simulink model "afe_rst_inv_psm_distributed_control_two_delays"  (R2026a)
settings: Solver=ode1be  StopTime=simlength  FixedStep=tc  MaxStep=Tc
values from neighbouring files (symbols this model uses):
  Amplitude_U = 1.16    [grid_fault_generator.m]
  Amplitude_V = Amplitude_U    (= 1.16)    [grid_fault_generator.m]
  Amplitude_W = Amplitude_U    (= 1.16)    [grid_fault_generator.m]
  end_time_LVRT = start_time_LVRT + error_length    [grid_fault_generator.m]
  Igrid_phase_normalization_factor = 270*sqrt(2)    [grid_emulator.m]
  omega_grid_emulator_nom = w_grid    (= 314.159265359)    [grid_emulator.m]
  omega_grid_nom = w_grid    (= 314.159265359)    [grid_emulator.m]
  t_ramp = 20e-3    (= 0.02)    [grid_fault_generator.m]
  ugrid_factor = 1    [grid_emulator.m]
  V_phase_normalization_factor = Vgrid_phase_normalization_factor    [grid_emulator.m]
  Vdc_bez = 1070    [grid_emulator.m]
  Vemu_ref_norm = Vemu_ref * sqrt(2) / V_phase_normalization_factor    [grid_emulator.m]
  vn_eta_pu = 0    [grid_emulator.m]
  vn_xi_pu = 0    [grid_emulator.m]
  vp_xi_pu = 1    [grid_emulator.m]
undefined symbols (not defined in the file or in its folder): Adrso, Aresd, Bresd, CFi, CFu, Cresd, Crso, CTRPIFF_CLIP_RELEASE, dead_time_INV, emf_fb_p, emf_fb_p_ccaller_1, emf_fb_p_ccaller_2, emf_p, emf_p_ccaller_1, emf_p_ccaller_2, fPWM_INV, g0_161Hz, g0_500Hz, g1_161Hz, g1_500Hz, i_grid_neg_eta_lim, i_grid_neg_eta_red_lim, i_grid_neg_xi_lim, i_grid_neg_xi_red_lim, i_grid_pos_eta_lim, i_grid_pos_eta_red_lim, ibez, id_lim, ieta_neg_ref_lim, ieta_pos_ref_lim, iq_lim, ixi_pos_ref_lim, Jm_norm, k_frt_ref, kg, ki_afe, ki_i, ki_id, ki_iq, ki_rc_neg_grid, ki_rc_pos_grid, ki_vs, ki_w, kp_afe, kp_i, kp_id, kp_iq, kp_rc_neg_grid, kp_rc_pos_grid, kp_vs, kp_w, kw, l1, l2, Lalpha_norm, Ld_norm, Ldrso, Lq_norm, Ls_norm, luenberger_l1 ... (+30)
libraries: fl_lib x146, nesl_utility x62, simulink x8, cstblocks_lti x7, sl_discontinuities x3, single_phase_transformer_lib x3, flexshaft_lib x1, permanent_magnet_synchronous_machine x1
(part 2 of 14)

== system afe_rst_inv_psm_distributed_control_two_delays/INV-Modular/threephase_vi_measures ==
  Bus Creator : BusCreator  Inputs=6
  Bus Selector : BusSelector  OutputSignals=usu,usv,usw  OutputAsBus=on
  Bus Selector1 : BusSelector  OutputSignals=isu,iuv,isw  OutputAsBus=on
  Current Sensor : fl_lib/Electrical/Electrical Sensors/Current Sensor
  Current Sensor1 : fl_lib/Electrical/Electrical Sensors/Current Sensor
  Current Sensor2 : fl_lib/Electrical/Electrical Sensors/Current Sensor
  Electrical Reference1 : fl_lib/Electrical/Electrical Elements/Electrical Reference
  Voltage Sensor : fl_lib/Electrical/Electrical Sensors/Voltage Sensor
  Voltage Sensor1 : fl_lib/Electrical/Electrical Sensors/Voltage Sensor
  Voltage Sensor2 : fl_lib/Electrical/Electrical Sensors/Voltage Sensor
  is_uvw/us_uvw : Scope  NumInputPorts=2
      settings: SampleTime=tc  ActiveDisplayYMinimum=-1567.0761  ActiveDisplayYMaximum=1567.45951  DataLoggingVariableName=ScopeData2
  isu_motor : nesl_utility/PS-Simulink Converter  PhysicalDomain=network_engine_domain  SubClassName=ps_output  LeftPortType=input  RightPortType=output  PseudoPeriodic=off  Frequencies=[]  VectorFormat=1-D array  Unit=A  AffineConversion=off
  isv_motor : nesl_utility/PS-Simulink Converter  PhysicalDomain=network_engine_domain  SubClassName=ps_output  LeftPortType=input  RightPortType=output  PseudoPeriodic=off  Frequencies=[]  VectorFormat=1-D array  Unit=A  AffineConversion=off
  isw_motor : nesl_utility/PS-Simulink Converter  PhysicalDomain=network_engine_domain  SubClassName=ps_output  LeftPortType=input  RightPortType=output  PseudoPeriodic=off  Frequencies=[]  VectorFormat=1-D array  Unit=A  AffineConversion=off
  uc_grid : nesl_utility/PS-Simulink Converter  PhysicalDomain=network_engine_domain  SubClassName=ps_output  LeftPortType=input  RightPortType=output  PseudoPeriodic=off  Frequencies=[]  VectorFormat=1-D array  Unit=V  AffineConversion=off
  usu_motor : nesl_utility/PS-Simulink Converter  PhysicalDomain=network_engine_domain  SubClassName=ps_output  LeftPortType=input  RightPortType=output  PseudoPeriodic=off  Frequencies=[]  VectorFormat=1-D array  Unit=V  AffineConversion=off
  usv_motor : nesl_utility/PS-Simulink Converter  PhysicalDomain=network_engine_domain  SubClassName=ps_output  LeftPortType=input  RightPortType=output  PseudoPeriodic=off  Frequencies=[]  VectorFormat=1-D array  Unit=V  AffineConversion=off
  Uu : PMIOPort  Side=Left
  uu : PMIOPort  Port=2  Side=Right
  Uv : PMIOPort  Port=3  Side=Left
  uv : PMIOPort  Port=4  Side=Right
  Uw : PMIOPort  Port=5  Side=Left
  uw : PMIOPort  Port=6  Side=Right
  tag scope: is_uvw_motor=global, us_uvw_motor=global
  wires:
  Bus Creator/1 -> Bus Selector1/1, Bus Selector/1  "vi_data"
  Bus Selector/1 -> [us_uvw_motor]
  isv_motor/1 -> Bus Creator/5  "iuv"
  isu_motor/1 -> Bus Creator/4  "isu"
  isw_motor/1 -> Bus Creator/6  "isw"
  usu_motor/1 -> Bus Creator/1  "usu"
  usv_motor/1 -> Bus Creator/2  "usv"
  uc_grid/1 -> Bus Creator/3  "usw"
  Bus Selector1/1 -> [is_uvw_motor]
  [us_uvw_motor] -> is_uvw/us_uvw/1
  [is_uvw_motor] -> is_uvw/us_uvw/2
  connections:
  Current Sensor1/LConn1 -- Uv/RConn1 -- Voltage Sensor1/LConn1
  Electrical Reference1/LConn1 -- Voltage Sensor/RConn2 -- Voltage Sensor2/RConn2 -- Voltage Sensor1/RConn2
  Voltage Sensor/RConn1 -- usu_motor/LConn1
  Current Sensor/RConn2 -- uu/RConn1
  Voltage Sensor1/RConn1 -- usv_motor/LConn1
  Voltage Sensor2/LConn1 -- Current Sensor2/LConn1 -- Uw/RConn1
  Current Sensor/LConn1 -- Uu/RConn1 -- Voltage Sensor/LConn1
  Current Sensor1/RConn2 -- uv/RConn1
  Voltage Sensor2/RConn1 -- uc_grid/LConn1
  isv_motor/LConn1 -- Current Sensor1/RConn1
  isu_motor/LConn1 -- Current Sensor/RConn1
  isw_motor/LConn1 -- Current Sensor2/RConn1
  Current Sensor2/RConn2 -- uw/RConn1

== system afe_rst_inv_psm_distributed_control_two_delays/brake/switch_5 ==
  Diode : fl_lib/Electrical/Electrical Elements/Diode  Vf=Vgamma V  Ron=Ron Ohm  Goff=1e-8 1/Ohm  i_specify=off  i_priority=None  i=0 A  i_nominal_specify=off  i_nominal_value=1  i_nominal_unit=A  v_specify=off  v_priority=None  v=0 V  v_nominal_specify=off  v_nominal_value=1  v_nominal_unit=V
  Switch : fl_lib/Electrical/Electrical Elements/Switch  R_closed=Ron Ohm  G_open=1e-8 1/Ohm  Threshold=7.5  i_specify=off  i_priority=None  i=0 A  i_nominal_specify=off  i_nominal_value=1  i_nominal_unit=A  v_specify=off  v_priority=None  v=0 V  v_nominal_specify=off  v_nominal_value=1  v_nominal_unit=V
  G : PMIOPort  Side=Left
  C : PMIOPort  Port=2  Side=Left
  E : PMIOPort  Port=3  Side=Right
  connections:
  Switch/RConn2 -- C/RConn1 -- Diode/RConn1
  Switch/RConn1 -- G/RConn1
  Switch/LConn1 -- E/RConn1 -- Diode/LConn1

== system afe_rst_inv_psm_distributed_control_two_delays/brake/switch_6 ==
  Diode : fl_lib/Electrical/Electrical Elements/Diode  Vf=Vgamma V  Ron=Ron Ohm  Goff=1e-8 1/Ohm  i_specify=off  i_priority=None  i=0 A  i_nominal_specify=off  i_nominal_value=1  i_nominal_unit=A  v_specify=off  v_priority=None  v=0 V  v_nominal_specify=off  v_nominal_value=1  v_nominal_unit=V
  C : PMIOPort  Side=Left
  E : PMIOPort  Port=2  Side=Right
  connections:
  E/RConn1 -- Diode/LConn1
  C/RConn1 -- Diode/RConn1

== system afe_rst_inv_psm_distributed_control_two_delays/grid/grid_emulator ==
  3ph_YYg : Subsystem
  Controlled Voltage Source : fl_lib/Electrical/Electrical Sources/Controlled Voltage Source
  Controlled Voltage Source1 : fl_lib/Electrical/Electrical Sources/Controlled Voltage Source
  Controlled Voltage Source2 : fl_lib/Electrical/Electrical Sources/Controlled Voltage Source
  Electrical Reference : fl_lib/Electrical/Electrical Elements/Electrical Reference
  Simulink-PS Converter : nesl_utility/Simulink-PS Converter  PhysicalDomain=network_engine_domain  SubClassName=ps_input  LeftPortType=input  RightPortType=output  PseudoPeriodic=off  Frequencies=[]  NoiseDistribution=none  NoiseParameters=[]  Unit=V  AffineConversion=on  FilteringAndDerivatives=provide  SimscapeFilterOrder=1  InputFilterTimeConstant=0.001  UdotUserProvided=0
  Simulink-PS Converter1 : nesl_utility/Simulink-PS Converter  PhysicalDomain=network_engine_domain  SubClassName=ps_input  LeftPortType=input  RightPortType=output  PseudoPeriodic=off  Frequencies=[]  NoiseDistribution=none  NoiseParameters=[]  Unit=V  AffineConversion=on  FilteringAndDerivatives=provide  SimscapeFilterOrder=1  InputFilterTimeConstant=0.001  UdotUserProvided=0
  Simulink-PS Converter2 : nesl_utility/Simulink-PS Converter  PhysicalDomain=network_engine_domain  SubClassName=ps_input  LeftPortType=input  RightPortType=output  PseudoPeriodic=off  Frequencies=[]  NoiseDistribution=none  NoiseParameters=[]  Unit=V  AffineConversion=on  FilteringAndDerivatives=provide  SimscapeFilterOrder=1  InputFilterTimeConstant=0.001  UdotUserProvided=0
  Solver Configuration : nesl_utility/Solver Configuration  PhysicalDomain=network_engine_domain  SubClassName=solver  LeftPortType=input  RightPortType=generic  Tones=[]  Harmonics=[]  SimulateNoise=off  Profile=off  UseLocalSampling=off  EnableSwitchedLinearOptims=on  FrequencyDomain=off  UseCCode=off  RelTol=0.001  AbsTol=0.001  MinStep=1e-09  ToWorkspace=off  RevertToSquareIcSolve=off  NumHomotopyIterations=100  PhasorMode=off  PhasorModeNumHarmonics=1  ConsistencySolver=NEWTON_FTOL  CanonicalOrdering=UNORDERED  OptimizeIntermediates=UNOPTIMIZED  IndexReductionMethod=DerivativeReplacement  DoDC=off  ResidualTolerance=1e-09  ConsistencyTolSource=GLOBAL  ConsistencyAbsTol=0.001  ConsistencyRelTol=0.001  ConsistencyTolFactor=0.001  UseLocalSolver=on  LocalSolverChoice=NE_BACKWARD_EULER_ADVANCER  ResolveIndetEquations=on  FunctionEvalNumThread=1  LocalSolverSampleTime=tc  DoFixedCost=on  MaxNonlinIter=3  MaxModeIter=2  ComputeImpulses=off  ImpulseIterations=2  LinearAlgebra=auto  LinearAlgebraNumThread=0  EquationFormulation=NE_TIME_EF  DelaysMemoryBudget=1024  AutomaticFiltering=on  FilteringTimeConstant=0.001  PartitionStorageMethod=AS_NEEDED  PartitionMemoryBudget=1024  PartitionMethod=ROBUST  MultibodyUseLocalSolver=off  MultibodyLocalSolverChoice=ODE1  MultibodyLocalSolverSampleTime=0.001
  grid_emulator : Subsystem
  threephase_vi_measures : Subsystem
  u1 : PMIOPort  Side=Right
  u2 : PMIOPort  Port=2  Side=Right
  u3 : PMIOPort  Port=3  Side=Right
  wires:
  grid_emulator/2(Vmb) -> Simulink-PS Converter1/1
  grid_emulator/3(Vmc) -> Simulink-PS Converter2/1
  grid_emulator/1(Vma) -> Simulink-PS Converter/1
  connections:
  Simulink-PS Converter/RConn1 -- Controlled Voltage Source/RConn1
  Simulink-PS Converter1/RConn1 -- Controlled Voltage Source1/RConn1
  Simulink-PS Converter2/RConn1 -- Controlled Voltage Source2/RConn1
  Electrical Reference/LConn1 -- Solver Configuration/RConn1 -- Controlled Voltage Source/RConn2 -- Controlled Voltage Source1/RConn2 -- Controlled Voltage Source2/RConn2
  3ph_YYg/RConn1 -- u1/RConn1
  3ph_YYg/RConn2 -- u2/RConn1
  3ph_YYg/RConn3 -- u3/RConn1
  threephase_vi_measures/LConn1 -- Controlled Voltage Source/LConn1
  threephase_vi_measures/LConn2 -- Controlled Voltage Source1/LConn1
  threephase_vi_measures/LConn3 -- Controlled Voltage Source2/LConn1
  threephase_vi_measures/RConn1 -- 3ph_YYg/LConn1
  threephase_vi_measures/RConn2 -- 3ph_YYg/LConn2
  threephase_vi_measures/RConn3 -- 3ph_YYg/LConn3

== system afe_rst_inv_psm_distributed_control_two_delays/grid/instantaneus_power ==
  Vline : Inport
  Iline : Inport  Port=2
  Demux2 : Demux  Outputs=3
  Demux3 : Demux  Outputs=3
  Fcn1 : Fcn  Expr=u(1)/(sqrt(u(1)^2+u(2)^2))
  Gain2 : Gain  Gain=3/2
  Gain3 : Gain  Gain=3/2
  Mux1 : Mux  Inputs=2
  Product{,1..3} (4 alike) : Product  RndMeth=Zero
  Sum : Sum  Inputs=|++
  Sum1 : Sum  Inputs=|+-
  To Workspace1 : ToWorkspace  VariableName=va_line_rms_sim  SampleTime=ts_afe
      settings: MaxDataPoints=Ns_afe
  To Workspace2 : ToWorkspace  VariableName=vb_line_rms_sim  SampleTime=ts_afe
      settings: MaxDataPoints=Ns_afe
  To Workspace3 : ToWorkspace  VariableName=vc_line_rms_sim  SampleTime=ts_afe
      settings: MaxDataPoints=Ns_afe
  To Workspace4 : ToWorkspace  VariableName=ia_line_rms_sim  SampleTime=ts_afe
      settings: MaxDataPoints=Ns_afe
  To Workspace5 : ToWorkspace  VariableName=ib_line_rms_sim  SampleTime=ts_afe
      settings: MaxDataPoints=Ns_afe
  To Workspace6 : ToWorkspace  VariableName=ic_line_rms_sim  SampleTime=ts_afe
      settings: MaxDataPoints=Ns_afe
  To Workspace7 : ToWorkspace  VariableName=Pline_avg_sim  SampleTime=ts_afe
      settings: MaxDataPoints=Ns_afe
  To Workspace8 : ToWorkspace  VariableName=Qline_avg_sim  SampleTime=ts_afe
      settings: MaxDataPoints=Ns_afe
  abc2alphabeta : Subsystem
  "abc2alphabeta " : Subsystem
  moving_avarage : Subsystem
  moving_avarage1 : Subsystem
  rms : Subsystem
  rms1 : Subsystem
  rms2 : Subsystem
  rms3 : Subsystem
  rms4 : Subsystem
  rms5 : Subsystem
  tag scope: Pline_avg=global, Qline_avg=global, cos_phi_avg=global
  wires:
  Gain3/1 -> moving_avarage1/1(In), To Workspace8/1
  Gain2/1 -> moving_avarage/1(In), To Workspace7/1
  Demux2/1 -> abc2alphabeta/1(a), rms/1(In1)
  Vline/1 -> Demux2/1
  Iline/1 -> Demux3/1
  abc2alphabeta/2(vline_beta) -> Product1/1, Product2/1
  "abc2alphabeta "/2(i_line_beta) -> Product3/1, Product1/2
  abc2alphabeta/1(vline_alpha) -> Product/1, Product3/2
  "abc2alphabeta "/1(i_line_alpha) -> Product2/2, Product/2
  Product/1 -> Sum/1
  Product1/1 -> Sum/2
  Product2/1 -> Sum1/1
  Product3/1 -> Sum1/2
  Sum1/1 -> Gain3/1
  Sum/1 -> Gain2/1
  Demux2/2 -> abc2alphabeta/2(b), rms1/1(In1)
  Demux2/3 -> abc2alphabeta/3(c), rms2/1(In1)
  Demux3/1 -> "abc2alphabeta "/1(a), rms3/1(In1)
  Demux3/2 -> "abc2alphabeta "/2(b), rms4/1(In1)
  Demux3/3 -> rms5/1(In1), "abc2alphabeta "/3(c)
  moving_avarage/1(Mean) -> [Pline_avg]
  moving_avarage1/1(Mean) -> [Qline_avg]
  [Qline_avg] -> Mux1/2
  Mux1/1 -> Fcn1/1
  Fcn1/1 -> [cos_phi_avg]
  [Pline_avg] -> Mux1/1
  rms/1(Out1) -> To Workspace1/1
  rms2/1(Out1) -> To Workspace3/1
  rms1/1(Out1) -> To Workspace2/1
  rms5/1(Out1) -> To Workspace6/1
  rms4/1(Out1) -> To Workspace5/1
  rms3/1(Out1) -> To Workspace4/1

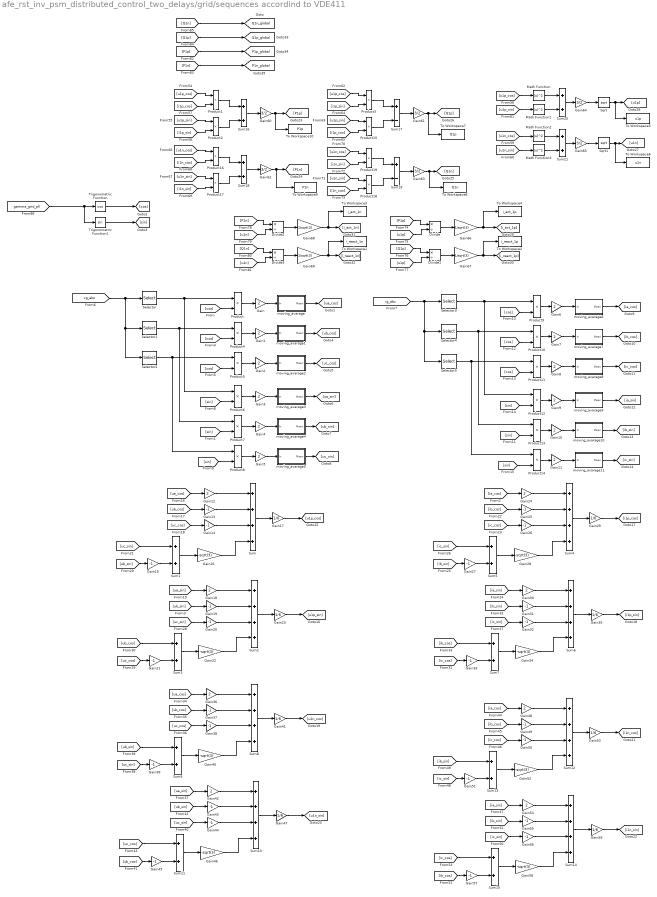
== system afe_rst_inv_psm_distributed_control_two_delays/grid/sequences accordind to VDE411 ==
  Divide{,1..3} (4 alike) : Product  Inputs=*/
  Gain{,1..12,18,24,30,36,42,48,54} (20 alike) : Gain  Gain=2
  Gain{13..15,19..21,25..27,31..33,37..39,43..45,49..51,55..57} (24 alike) : Gain  Gain=-1
  Gain{16,22,28,34,40,46,52,58} (8 alike) : Gain  Gain=-sqrt(3)
  Gain{17,23,29,35,41,47,53,59} (8 alike) : Gain  Gain=1/6
  Gain{60..65} (6 alike) : Gain  Gain=3/2
  Gain{66..69} (4 alike) : Gain  Gain=1/sqrt(3)
  Math Function{,1..3} (4 alike) : Math  Operator=magnitude^2  SignedPower=on
  Product{,1..19} (20 alike) : Product  RndMeth=Zero
  Selector : Selector  InputPortWidth=3  IndexOptions=Index vector (dialog)  Indices=1  OutputSizes=1
  Selector1 : Selector  InputPortWidth=3  IndexOptions=Index vector (dialog)  Indices=2  OutputSizes=1
  Selector2 : Selector  InputPortWidth=3  IndexOptions=Index vector (dialog)  Indices=3  OutputSizes=1
  Selector3 : Selector  InputPortWidth=3  IndexOptions=Index vector (dialog)  Indices=1  OutputSizes=1
  Selector4 : Selector  InputPortWidth=3  IndexOptions=Index vector (dialog)  Indices=2  OutputSizes=1
  Selector5 : Selector  InputPortWidth=3  IndexOptions=Index vector (dialog)  Indices=3  OutputSizes=1
  Sqrt : Sqrt
  Sqrt1 : Sqrt
  Sum{,2,4,6,8,10,12,14} (8 alike) : Sum  Inputs=++++
  Sum{1,3,5,7,9,11,13,15..16,18,20..21} (12 alike) : Sum
  Sum17 : Sum  Inputs=+-
  Sum19 : Sum  Inputs=+-
  To Workspace1 : ToWorkspace  VariableName=i_react_1n  SampleTime=ts_afe
      settings: MaxDataPoints=Ns_afe
  To Workspace10 : ToWorkspace  VariableName=P1p  SampleTime=ts_afe
      settings: MaxDataPoints=Ns_afe
  To Workspace2 : ToWorkspace  VariableName=i_react_1p  SampleTime=ts_afe
      settings: MaxDataPoints=Ns_afe
  To Workspace3 : ToWorkspace  VariableName=i_act_1n  SampleTime=ts_afe
      settings: MaxDataPoints=Ns_afe
  To Workspace4 : ToWorkspace  VariableName=i_act_1p  SampleTime=ts_afe
      settings: MaxDataPoints=Ns_afe
  To Workspace5 : ToWorkspace  VariableName=u1p  SampleTime=ts_afe
      settings: MaxDataPoints=Ns_afe
  To Workspace6 : ToWorkspace  VariableName=u1n  SampleTime=ts_afe
      settings: MaxDataPoints=Ns_afe
  To Workspace7 : ToWorkspace  VariableName=Q1p  SampleTime=ts_afe
      settings: MaxDataPoints=Ns_afe
  To Workspace8 : ToWorkspace  VariableName=Q1n  SampleTime=ts_afe
      settings: MaxDataPoints=Ns_afe
  To Workspace9 : ToWorkspace  VariableName=P1n  SampleTime=ts_afe
      settings: MaxDataPoints=Ns_afe
  Trigonometric Function : Trigonometry  Operator=cos
  Trigonometric Function1 : Trigonometry
  moving_avarage : Subsystem
  moving_avarage1 : Subsystem
  moving_avarage10 : Subsystem
  moving_avarage11 : Subsystem
  moving_avarage2 : Subsystem
  moving_avarage3 : Subsystem
  moving_avarage4 : Subsystem
  moving_avarage5 : Subsystem
  moving_avarage6 : Subsystem
  moving_avarage7 : Subsystem
  moving_avarage8 : Subsystem
  moving_avarage9 : Subsystem
  tag scope: P1n_global=global, P1p_global=global, Q1n_global=global, Q1p_global=global
  wires:
  [vg_abc] -> Selector2/1, Selector1/1, Selector/1
  Trigonometric Function1/1 -> [sin]
  Trigonometric Function/1 -> [cos]
  [gamma_grid_pll] -> Trigonometric Function/1, Trigonometric Function1/1
  [cos] -> Product/2
  Product/1 -> Gain/1
  [cos] -> Product4/2
  Product4/1 -> Gain1/1
  [cos] -> Product5/2
  Product5/1 -> Gain2/1
  [sin] -> Product6/2
  Selector/1 -> Product6/1, Product/1
  Product6/1 -> Gain3/1
  [sin] -> Product7/2
  Selector1/1 -> Product7/1, Product4/1
  Product7/1 -> Gain4/1
  [sin] -> Product8/2
  Selector2/1 -> Product8/1, Product5/1
  Product8/1 -> Gain5/1
  [ig_abc] -> Selector3/1, Selector4/1, Selector5/1
  [cos] -> Product9/2
  Product9/1 -> Gain6/1
  [cos] -> Product10/2
  Product10/1 -> Gain7/1
  [cos] -> Product11/2
  Product11/1 -> Gain8/1
  [sin] -> Product12/2
  Selector3/1 -> Product9/1, Product12/1
  Product12/1 -> Gain9/1
  [sin] -> Product13/2
  Selector4/1 -> Product10/1, Product13/1
  Product13/1 -> Gain10/1
  [sin] -> Product14/2
  Selector5/1 -> Product11/1, Product14/1
  Product14/1 -> Gain11/1
  Gain/1 -> moving_avarage/1(In)
  moving_avarage/1(Mean) -> [ua_cos]
  Gain1/1 -> moving_avarage1/1(In)
  Gain2/1 -> moving_avarage2/1(In)
  Gain3/1 -> moving_avarage3/1(In)
  Gain4/1 -> moving_avarage4/1(In)
  Gain5/1 -> moving_avarage5/1(In)
  Gain6/1 -> moving_avarage6/1(In)
  Gain7/1 -> moving_avarage7/1(In)
  Gain8/1 -> moving_avarage8/1(In)
  Gain9/1 -> moving_avarage9/1(In)
  Gain10/1 -> moving_avarage10/1(In)
  Gain11/1 -> moving_avarage11/1(In)
  [ua_cos] -> Gain12/1
  [ub_cos] -> Gain13/1
  [uc_cos] -> Gain14/1
  [uc_sin] -> Sum1/1
  Gain15/1 -> Sum1/2
  [ub_sin] -> Gain15/1
  Sum1/1 -> Gain16/1
  Gain16/1 -> Sum/4
  Gain14/1 -> Sum/3
  Gain13/1 -> Sum/2
  Gain12/1 -> Sum/1
  Sum/1 -> Gain17/1
  Gain17/1 -> [u1p_cos]
  [ua_sin] -> Gain18/1
  [ub_sin] -> Gain19/1
  [uc_sin] -> Gain20/1
  [ub_cos] -> Sum3/1
  Gain21/1 -> Sum3/2
  [uc_cos] -> Gain21/1
  Sum3/1 -> Gain22/1
  Gain22/1 -> Sum2/4
  Gain20/1 -> Sum2/3
  Gain19/1 -> Sum2/2
  Gain18/1 -> Sum2/1
  Sum2/1 -> Gain23/1
  Gain23/1 -> [u1p_sin]
  [ia_cos] -> Gain24/1
  [ib_cos] -> Gain25/1
  [ic_cos] -> Gain26/1
  [ic_sin] -> Sum5/1
  Gain27/1 -> Sum5/2
  [ib_sin] -> Gain27/1
  Sum5/1 -> Gain28/1
  Gain28/1 -> Sum4/4
  Gain26/1 -> Sum4/3
  Gain25/1 -> Sum4/2
  Gain24/1 -> Sum4/1
  Sum4/1 -> Gain29/1
  Gain29/1 -> [i1p_cos]
  [ia_sin] -> Gain30/1
  [ib_sin] -> Gain31/1
  [ic_sin] -> Gain32/1
  [ib_cos] -> Sum7/1
  Gain33/1 -> Sum7/2
  [ic_cos] -> Gain33/1
  Sum7/1 -> Gain34/1
  Gain34/1 -> Sum6/4
  Gain32/1 -> Sum6/3
  Gain31/1 -> Sum6/2
  Gain30/1 -> Sum6/1
  Sum6/1 -> Gain35/1
  Gain35/1 -> [i1p_sin]
  [ua_cos] -> Gain36/1
  [ub_cos] -> Gain37/1
  [uc_cos] -> Gain38/1
  [ub_sin] -> Sum9/1
  Gain39/1 -> Sum9/2
  [uc_sin] -> Gain39/1
  Sum9/1 -> Gain40/1
  Gain40/1 -> Sum8/4
  Gain38/1 -> Sum8/3
  Gain37/1 -> Sum8/2
  Gain36/1 -> Sum8/1
  Sum8/1 -> Gain41/1
  Gain41/1 -> [u1n_cos]
  [ua_sin] -> Gain42/1
  [ub_sin] -> Gain43/1
  [uc_sin] -> Gain44/1
  [uc_cos] -> Sum11/1
  Gain45/1 -> Sum11/2
  [ub_cos] -> Gain45/1
  Sum11/1 -> Gain46/1
  Gain46/1 -> Sum10/4
  Gain44/1 -> Sum10/3
  Gain43/1 -> Sum10/2
  Gain42/1 -> Sum10/1
  Sum10/1 -> Gain47/1
  Gain47/1 -> [u1n_sin]
  [ia_cos] -> Gain48/1
  [ib_cos] -> Gain49/1
  [ic_cos] -> Gain50/1
  [ib_sin] -> Sum13/1
  Gain51/1 -> Sum13/2
  [ic_sin] -> Gain51/1
  Sum13/1 -> Gain52/1
  Gain52/1 -> Sum12/4
  Gain50/1 -> Sum12/3
  Gain49/1 -> Sum12/2
  Gain48/1 -> Sum12/1
  Sum12/1 -> Gain53/1
  Gain53/1 -> [i1n_cos]
  [ia_sin] -> Gain54/1
  [ib_sin] -> Gain55/1
  [ic_sin] -> Gain56/1
  [ic_cos] -> Sum15/1
  Gain57/1 -> Sum15/2
  [ib_cos] -> Gain57/1
  Sum15/1 -> Gain58/1
  Gain58/1 -> Sum14/4
  Gain56/1 -> Sum14/3
  Gain55/1 -> Sum14/2
  Gain54/1 -> Sum14/1
  Sum14/1 -> Gain59/1
  Gain59/1 -> [i1n_sin]
  Sum16/1 -> Gain60/1
  Product1/1 -> Sum16/1
  Product2/1 -> Sum16/2
  Gain60/1 -> To Workspace10/1, [P1p]
  [u1p_cos] -> Product1/1
  [i1p_cos] -> Product1/2
  [u1p_sin] -> Product2/1
  [i1p_sin] -> Product2/2
  Sum17/1 -> Gain61/1
  Product3/1 -> Sum17/1
  Product15/1 -> Sum17/2
  Gain61/1 -> To Workspace7/1, [Q1p]
  [u1p_cos] -> Product3/1
  [i1p_sin] -> Product3/2
  [u1p_sin] -> Product15/1
  [i1p_cos] -> Product15/2
  Sum18/1 -> Gain62/1
  Product16/1 -> Sum18/1
  Product17/1 -> Sum18/2
  Gain62/1 -> To Workspace9/1, [P1n]
  [u1n_cos] -> Product16/1
  [i1n_cos] -> Product16/2
  [u1n_sin] -> Product17/1
  [i1n_sin] -> Product17/2
  Sum19/1 -> Gain63/1
  Product19/1 -> Sum19/1
  Product18/1 -> Sum19/2
  Gain63/1 -> To Workspace8/1, [Q1n]
  [u1n_cos] -> Product19/1
  [i1n_sin] -> Product19/2
  [u1n_sin] -> Product18/1
  [i1n_cos] -> Product18/2
  [u1p_cos] -> Math Function/1
  [u1p_sin] -> Math Function1/1
  Math Function/1 -> Sum20/1
  Math Function1/1 -> Sum20/2
  Sum20/1 -> Gain64/1
  Gain64/1 -> Sqrt/1
  Sqrt/1 -> To Workspace5/1, [u1p]
  [u1n_cos] -> Math Function2/1
  [u1n_sin] -> Math Function3/1
  Math Function2/1 -> Sum21/1
  Math Function3/1 -> Sum21/2
  Sum21/1 -> Gain65/1
  Gain65/1 -> Sqrt1/1
  Sqrt1/1 -> To Workspace6/1, [u1n]
  [P1p] -> Divide/1
  [u1p] -> Divide/2
  Divide/1 -> Gain66/1
  Gain66/1 -> To Workspace4/1, [i_act_1p]
  [Q1p] -> Divide1/1
  [u1p] -> Divide1/2
  Divide1/1 -> Gain67/1
  Gain67/1 -> To Workspace2/1, [i_react_1p]
  [P1n] -> Divide2/1
  [u1n] -> Divide2/2
  Divide2/1 -> Gain68/1
  Gain68/1 -> To Workspace3/1, [i_act_1n]
  [Q1n] -> Divide3/1
  [u1n] -> Divide3/2
  Divide3/1 -> Gain69/1
  Gain69/1 -> To Workspace1/1, [i_react_1n]
  moving_avarage1/1(Mean) -> [ub_cos]
  moving_avarage2/1(Mean) -> [uc_cos]
  moving_avarage3/1(Mean) -> [ua_sin]
  moving_avarage4/1(Mean) -> [ub_sin]
  moving_avarage5/1(Mean) -> [uc_sin]
  moving_avarage6/1(Mean) -> [ia_cos]
  moving_avarage7/1(Mean) -> [ib_cos]
  moving_avarage8/1(Mean) -> [ic_cos]
  moving_avarage9/1(Mean) -> [ia_sin]
  moving_avarage10/1(Mean) -> [ib_sin]
  moving_avarage11/1(Mean) -> [ic_sin]
  [Q1n] -> [Q1n_global]
  [Q1p] -> [Q1p_global]
  [P1p] -> [P1p_global]
  [P1n] -> [P1n_global]

== system afe_rst_inv_psm_distributed_control_two_delays/grid/threephase_vi_measures ==
  Bus Creator : BusCreator  Inputs=6
  Bus Selector : BusSelector  OutputSignals=ua,ub,uc  OutputAsBus=on
  Bus Selector1 : BusSelector  OutputSignals=iga,igb,igc  OutputAsBus=on
  Current Sensor : fl_lib/Electrical/Electrical Sensors/Current Sensor
  Current Sensor1 : fl_lib/Electrical/Electrical Sensors/Current Sensor
  Current Sensor2 : fl_lib/Electrical/Electrical Sensors/Current Sensor
  Electrical Reference1 : fl_lib/Electrical/Electrical Elements/Electrical Reference
  Voltage Sensor : fl_lib/Electrical/Electrical Sensors/Voltage Sensor
  Voltage Sensor1 : fl_lib/Electrical/Electrical Sensors/Voltage Sensor
  Voltage Sensor2 : fl_lib/Electrical/Electrical Sensors/Voltage Sensor
  ia_grid : nesl_utility/PS-Simulink Converter  PhysicalDomain=network_engine_domain  SubClassName=ps_output  LeftPortType=input  RightPortType=output  PseudoPeriodic=off  Frequencies=[]  VectorFormat=1-D array  Unit=A  AffineConversion=off
  ib_grid : nesl_utility/PS-Simulink Converter  PhysicalDomain=network_engine_domain  SubClassName=ps_output  LeftPortType=input  RightPortType=output  PseudoPeriodic=off  Frequencies=[]  VectorFormat=1-D array  Unit=A  AffineConversion=off
  ic_grid : nesl_utility/PS-Simulink Converter  PhysicalDomain=network_engine_domain  SubClassName=ps_output  LeftPortType=input  RightPortType=output  PseudoPeriodic=off  Frequencies=[]  VectorFormat=1-D array  Unit=A  AffineConversion=off
  ig_abc/ug_abc : Scope  NumInputPorts=2
      settings: SampleTime=tc  ActiveDisplayYMinimum=-781.63744  ActiveDisplayYMaximum=887.15685  DataLoggingVariableName=ScopeData2
  ua_grid : nesl_utility/PS-Simulink Converter  PhysicalDomain=network_engine_domain  SubClassName=ps_output  LeftPortType=input  RightPortType=output  PseudoPeriodic=off  Frequencies=[]  VectorFormat=1-D array  Unit=V  AffineConversion=off
  ub_grid : nesl_utility/PS-Simulink Converter  PhysicalDomain=network_engine_domain  SubClassName=ps_output  LeftPortType=input  RightPortType=output  PseudoPeriodic=off  Frequencies=[]  VectorFormat=1-D array  Unit=V  AffineConversion=off
  uc_grid : nesl_utility/PS-Simulink Converter  PhysicalDomain=network_engine_domain  SubClassName=ps_output  LeftPortType=input  RightPortType=output  PseudoPeriodic=off  Frequencies=[]  VectorFormat=1-D array  Unit=V  AffineConversion=off
  Ua : PMIOPort  Side=Left
  ua : PMIOPort  Port=2  Side=Right
  Ub : PMIOPort  Port=3  Side=Left
  ub : PMIOPort  Port=4  Side=Right
  Uc : PMIOPort  Port=5  Side=Left
  uc : PMIOPort  Port=6  Side=Right
  tag scope: ig_abc=global, vg_abc=global
  wires:
  Bus Creator/1 -> Bus Selector1/1, Bus Selector/1  "vi_data"
  Bus Selector/1 -> [vg_abc]
  ib_grid/1 -> Bus Creator/5  "igb"
  ia_grid/1 -> Bus Creator/4  "iga"
  ic_grid/1 -> Bus Creator/6  "igc"
  ua_grid/1 -> Bus Creator/1  "ua"
  ub_grid/1 -> Bus Creator/2  "ub"
  uc_grid/1 -> Bus Creator/3  "uc"
  Bus Selector1/1 -> [ig_abc]
  [vg_abc] -> ig_abc/ug_abc/2
  [ig_abc] -> ig_abc/ug_abc/1
  connections:
  Current Sensor1/LConn1 -- ub/RConn1 -- Voltage Sensor1/LConn1
  Electrical Reference1/LConn1 -- Voltage Sensor/RConn2 -- Voltage Sensor2/RConn2 -- Voltage Sensor1/RConn2
  Voltage Sensor/RConn1 -- ua_grid/LConn1
  Ua/RConn1 -- Current Sensor/RConn2
  Voltage Sensor1/RConn1 -- ub_grid/LConn1
  Voltage Sensor2/LConn1 -- uc/RConn1 -- Current Sensor2/LConn1
  Current Sensor/LConn1 -- ua/RConn1 -- Voltage Sensor/LConn1
  Ub/RConn1 -- Current Sensor1/RConn2
  Voltage Sensor2/RConn1 -- uc_grid/LConn1
  ib_grid/LConn1 -- Current Sensor1/RConn1
  ia_grid/LConn1 -- Current Sensor/RConn1
  ic_grid/LConn1 -- Current Sensor2/RConn1
  Uc/RConn1 -- Current Sensor2/RConn2

== system afe_rst_inv_psm_distributed_control_two_delays/grid filter/threephase_vi_measures_stack ==
  Bus Creator : BusCreator  Inputs=6
  Current Sensor : fl_lib/Electrical/Electrical Sensors/Current Sensor
  Current Sensor1 : fl_lib/Electrical/Electrical Sensors/Current Sensor
  Current Sensor2 : fl_lib/Electrical/Electrical Sensors/Current Sensor
  Electrical Reference1 : fl_lib/Electrical/Electrical Elements/Electrical Reference
  Selector : Selector  InputPortWidth=6  IndexOptions=Index vector (dialog)  Indices=[1 2 3]  OutputSizes=1
  Selector1 : Selector  InputPortWidth=6  IndexOptions=Index vector (dialog)  Indices=[4 5 6]  OutputSizes=1
  Voltage Sensor : fl_lib/Electrical/Electrical Sensors/Voltage Sensor
  Voltage Sensor1 : fl_lib/Electrical/Electrical Sensors/Voltage Sensor
  Voltage Sensor2 : fl_lib/Electrical/Electrical Sensors/Voltage Sensor
  ia_afe : nesl_utility/PS-Simulink Converter  PhysicalDomain=network_engine_domain  SubClassName=ps_output  LeftPortType=input  RightPortType=output  PseudoPeriodic=off  Frequencies=[]  VectorFormat=1-D array  Unit=A  AffineConversion=off
  ib_afe : nesl_utility/PS-Simulink Converter  PhysicalDomain=network_engine_domain  SubClassName=ps_output  LeftPortType=input  RightPortType=output  PseudoPeriodic=off  Frequencies=[]  VectorFormat=1-D array  Unit=A  AffineConversion=off
  ic_afe : nesl_utility/PS-Simulink Converter  PhysicalDomain=network_engine_domain  SubClassName=ps_output  LeftPortType=input  RightPortType=output  PseudoPeriodic=off  Frequencies=[]  VectorFormat=1-D array  Unit=A  AffineConversion=off
  is_abc/us_abc : Scope  NumInputPorts=2
      settings: SampleTime=tc  ActiveDisplayYMinimum=-168.28271  ActiveDisplayYMaximum=145.46709
  ua_afe : nesl_utility/PS-Simulink Converter  PhysicalDomain=network_engine_domain  SubClassName=ps_output  LeftPortType=input  RightPortType=output  PseudoPeriodic=off  Frequencies=[]  VectorFormat=1-D array  Unit=V  AffineConversion=off
  ub_afe : nesl_utility/PS-Simulink Converter  PhysicalDomain=network_engine_domain  SubClassName=ps_output  LeftPortType=input  RightPortType=output  PseudoPeriodic=off  Frequencies=[]  VectorFormat=1-D array  Unit=V  AffineConversion=off
  uc_afe : nesl_utility/PS-Simulink Converter  PhysicalDomain=network_engine_domain  SubClassName=ps_output  LeftPortType=input  RightPortType=output  PseudoPeriodic=off  Frequencies=[]  VectorFormat=1-D array  Unit=V  AffineConversion=off
  Ua : PMIOPort  Side=Left
  ua : PMIOPort  Port=2  Side=Right
  Ub : PMIOPort  Port=3  Side=Left
  ub : PMIOPort  Port=4  Side=Right
  Uc : PMIOPort  Port=5  Side=Left
  uc : PMIOPort  Port=6  Side=Right
  tag scope: is_abc=global, vs_abc=global
  wires:
  Bus Creator/1 -> Selector1/1, Selector/1  "vi_data"
  Selector/1 -> [vs_abc]
  ib_afe/1 -> Bus Creator/5  "ib_afe"
  ia_afe/1 -> Bus Creator/4  "ia_afe"
  ic_afe/1 -> Bus Creator/6  "ic_afe"
  ua_afe/1 -> Bus Creator/1  "ua_afe"
  ub_afe/1 -> Bus Creator/2  "ub_afe"
  uc_afe/1 -> Bus Creator/3  "uc_afe"
  Selector1/1 -> [is_abc]
  [is_abc] -> is_abc/us_abc/1
  [vs_abc] -> is_abc/us_abc/2
  connections:
  Current Sensor1/LConn1 -- Voltage Sensor1/LConn1 -- Ub/RConn1
  Electrical Reference1/LConn1 -- Voltage Sensor1/RConn2 -- Voltage Sensor2/RConn2 -- Voltage Sensor/RConn2
  Voltage Sensor/RConn1 -- ua_afe/LConn1
  Current Sensor/RConn2 -- ua/RConn1
  Voltage Sensor1/RConn1 -- ub_afe/LConn1
  Voltage Sensor2/LConn1 -- Uc/RConn1 -- Current Sensor2/LConn1
  Current Sensor/LConn1 -- Voltage Sensor/LConn1 -- Ua/RConn1
  Current Sensor1/RConn2 -- ub/RConn1
  Voltage Sensor2/RConn1 -- uc_afe/LConn1
  ib_afe/LConn1 -- Current Sensor1/RConn1
  ia_afe/LConn1 -- Current Sensor/RConn1
  ic_afe/LConn1 -- Current Sensor2/RConn1
  Current Sensor2/RConn2 -- uc/RConn1

== system afe_rst_inv_psm_distributed_control_two_delays/mainboard_afe/current_sequence_avg ==
  i_grid_pos_xi : Inport
  i_grid_pos_eta : Inport  Port=2
  i_grid_neg_xi : Inport  Port=3
  i_grid_neg_eta : Inport  Port=4
  Moving Average Filter5 : Subsystem
  Moving Average Filter6 : Subsystem
  Moving Average Filter7 : Subsystem
  Moving Average Filter8 : Subsystem
  i_grid_pos_xi_avg : Outport
  i_grid_pos_eta_avg : Outport  Port=2
  i_grid_neg_xi_avg : Outport  Port=3
  i_grid_neg_eta_avg : Outport  Port=4
  wires:
  [omega_grid_pll] -> Moving Average Filter5/2(In3), Moving Average Filter6/2(In3), Moving Average Filter7/2(In3), Moving Average Filter8/2(In3)
  Moving Average Filter8/1(xi) -> i_grid_neg_eta_avg/1
  i_grid_neg_eta/1 -> Moving Average Filter8/1(In2)
  i_grid_neg_xi/1 -> Moving Average Filter7/1(In2)
  Moving Average Filter7/1(xi) -> i_grid_neg_xi_avg/1
  Moving Average Filter6/1(xi) -> i_grid_pos_eta_avg/1
  i_grid_pos_eta/1 -> Moving Average Filter6/1(In2)
  i_grid_pos_xi/1 -> Moving Average Filter5/1(In2)
  Moving Average Filter5/1(xi) -> i_grid_pos_xi_avg/1

== system afe_rst_inv_psm_distributed_control_two_delays/mainboard_afe/dq_pll ==
  note: SRF-PLL
  phase_pll/phase_grid : Scope  NumInputPorts=2
      settings: SampleTime=ts_afe  ActiveDisplayYMinimum=-3.92699  ActiveDisplayYMaximum=3.92699
  pll_stageA : Subsystem
  pll_stageB : Subsystem
  tag scope: gamma_grid_pll=global
  wires:
  pll_stageB/1(gamma_grid_pll) -> pll_stageA/1(gamma_grid), phase_pll/phase_grid/1, [gamma_grid_pll]
  pll_stageA/2(u_grid_pos_eta) -> pll_stageB/2(u_grid_pos_eta)  "u_grid_pos_eta"
  pll_stageA/1(u_grid_pos_xi) -> pll_stageB/1(u_grid_pos_xi)  "u_grid_pos_xi"
  [gamma_grid_emulator] -> phase_pll/phase_grid/2

== system afe_rst_inv_psm_distributed_control_two_delays/mainboard_afe/grid_current_sampling_and_alpha_beta_transformation ==
  Mux : Mux  Inputs=3
  Selector : Selector  InputPortWidth=3  IndexOptions=Index vector (dialog)  Indices=1  OutputSizes=1
  i_abc2alphabeta : MATLAB Function  TreatAsAtomicUnit=on  SystemSampleTime=ts_afe
  ig_hat/ig : Scope  NumInputPorts=2
      settings: SampleTime=tc  ActiveDisplayYMinimum=-1.06426  ActiveDisplayYMaximum=1.44682  DataLoggingVariableName=ScopeData2
  ig_hat/ig1 : Scope  NumInputPorts=2
      settings: SampleTime=tc  ActiveDisplayYMinimum=-2.36968  ActiveDisplayYMaximum=2.03597  DataLoggingVariableName=ScopeData3
  iga_measure : Subsystem
  i_grid_alpha : Outport
  i_grid_beta : Outport  Port=2
  wires:
  i_abc2alphabeta/2(beta) -> i_grid_beta/1  "i_grid_beta"
  i_abc2alphabeta/1(alpha) -> i_grid_alpha/1  "i_grid_alpha"
  [ig_abc] -> iga_measure/1(ig)
  [iga_pu_dba_fb_mbafe] -> Mux/1
  [igb_pu_dbb_fb_mbafe] -> Mux/2
  [igc_pu_dbc_fb_mbafe] -> Mux/3
  Mux/1 -> ig_hat/ig1/1
  iga_measure/1(ig_pu) -> i_abc2alphabeta/1(i_abc), Selector/1, ig_hat/ig1/2
  [iga_pu_dba] -> ig_hat/ig/1
  Selector/1 -> ig_hat/ig/2

== system afe_rst_inv_psm_distributed_control_two_delays/mainboard_afe/grid_voltage_sampling_and_alpha_beta_transformation ==
  Mux : Mux  Inputs=3
  v_abc2alphabeta : MATLAB Function  TreatAsAtomicUnit=on  SystemSampleTime=ts_afe
  u_grid_alpha : Outport
  u_grid_beta : Outport  Port=2
  wires:
  v_abc2alphabeta/1(alpha) -> u_grid_alpha/1  "u_grid_alpha"
  v_abc2alphabeta/2(beta) -> u_grid_beta/1  "u_grid_beta"
  Mux/1 -> v_abc2alphabeta/1(v_abc)
  [uga_pu_dba_fb_mbafe] -> Mux/1
  [ugb_pu_dbb_fb_mbafe] -> Mux/2
  [ugc_pu_dbc_fb_mbafe] -> Mux/3

== system afe_rst_inv_psm_distributed_control_two_delays/mainboard_afe/ig_alphabeta2xieta ==
  alpha : Inport
  beta : Inport  Port=2
  gamma : Inport  Port=3
  MATLAB Function : MATLAB Function  TreatAsAtomicUnit=on
  MATLAB Function1 : MATLAB Function  TreatAsAtomicUnit=on
  xi : Outport
  v_grid_pos_eta : Outport  Port=2
  v_grid_neg_xi : Outport  Port=3
  e : Outport  Port=4
  wires:
  alpha/1 -> MATLAB Function1/1(alpha), MATLAB Function/1(alpha)  "i_grid_alpha"
  beta/1 -> MATLAB Function1/2(beta), MATLAB Function/2(beta)  "i_grid_beta"
  gamma/1 -> MATLAB Function1/3(gamma), MATLAB Function/3(gamma)  "gamma_grid"
  MATLAB Function/2(eta) -> v_grid_pos_eta/1  "i_grid_pos_eta"
  MATLAB Function1/1(xi) -> v_grid_neg_xi/1  "i_grid_neg_xi"
  MATLAB Function1/2(eta) -> e/1  "i_grid_neg_eta"
  MATLAB Function/1(xi) -> xi/1  "i_grid_pos_xi"

== system afe_rst_inv_psm_distributed_control_two_delays/mainboard_afe/sequences_current_control ==
  i_pos_xi : Inport
  i_pos_eta : Inport  Port=2
  i_neg_xi : Inport  Port=3
  i_neg_eta : Inport  Port=4
  Bus Selector : BusSelector  OutputSignals=i_grid_pos_eta_ref,i_grid_neg_eta_ref,i_grid_neg_xi_ref
  Constant3 : Constant  Value=0
  Constant4 : Constant  Value=0
  Constant5 : Constant  Value=0
  Sum : Sum  Inputs=|+-
  Sum1 : Sum  Inputs=|+-
  Sum2 : Sum  Inputs=|+-
  Terminator : Terminator
  negative_sequence_eta_current_control : Subsystem
  negative_sequence_xi_current_control : Subsystem
  positive_sequence_eta_current_control : Subsystem
  tag scope: i_stack_neg_eta_ref=global, i_stack_neg_xi_ref=global, i_stack_pos_eta_ref=global
  wires:
  i_pos_xi/1 -> Terminator/1
  [i_grid_seq_ref] -> Bus Selector/1
  Bus Selector/1 -> Sum/1  "<i_grid_pos_eta_ref>"
  Bus Selector/2 -> Sum1/1  "<i_grid_neg_eta_ref>"
  Bus Selector/3 -> Sum2/1  "<i_grid_neg_xi_ref>"
  i_pos_eta/1 -> Sum/2
  i_neg_eta/1 -> Sum1/2
  i_neg_xi/1 -> Sum2/2
  Constant3/1 -> positive_sequence_eta_current_control/1(ff)
  Constant4/1 -> negative_sequence_eta_current_control/1(ff)
  Constant5/1 -> negative_sequence_xi_current_control/1(ff)
  negative_sequence_xi_current_control/1(u) -> [i_stack_neg_xi_ref]
  negative_sequence_eta_current_control/1(u) -> [i_stack_neg_eta_ref]
  positive_sequence_eta_current_control/1(u) -> [i_stack_pos_eta_ref]
  Sum/1 -> positive_sequence_eta_current_control/2(e)
  Sum1/1 -> negative_sequence_eta_current_control/2(e)
  Sum2/1 -> negative_sequence_xi_current_control/2(e)

== system afe_rst_inv_psm_distributed_control_two_delays/mainboard_afe/ug_alphabeta2xieta ==
  alpha : Inport
  beta : Inport  Port=2
  gamma : Inport  Port=3
  MATLAB Function : MATLAB Function  TreatAsAtomicUnit=on
  MATLAB Function1 : MATLAB Function  TreatAsAtomicUnit=on
  xi : Outport
  eta : Outport  Port=2
  v_grid_neg_xi : Outport  Port=3
  v_grid_neg_eta : Outport  Port=4
  wires:
  alpha/1 -> MATLAB Function1/1(alpha), MATLAB Function/1(alpha)  "u_grid_alpha"
  beta/1 -> MATLAB Function1/2(beta), MATLAB Function/2(beta)  "u_grid_beta"
  gamma/1 -> MATLAB Function1/3(gamma), MATLAB Function/3(gamma)  "gamma_grid"
  MATLAB Function/1(xi) -> xi/1  "u_grid_pos_xi"
  MATLAB Function/2(eta) -> eta/1  "u_grid_pos_eta"
  MATLAB Function1/1(xi) -> v_grid_neg_xi/1  "u_grid_neg_xi"
  MATLAB Function1/2(eta) -> v_grid_neg_eta/1  "u_grid_neg_eta"

== system afe_rst_inv_psm_distributed_control_two_delays/mainboard_afe/voltage-current-acquisition ==
  iga_fieldbus : Subsystem
  igb_fieldbus : Subsystem
  igc_fieldbus : Subsystem
  isa_fieldbus : Subsystem
  isb_fieldbus : Subsystem
  isc_fieldbus : Subsystem
  uga_fieldbus : Subsystem
  ugb_fieldbus : Subsystem
  ugb_fieldbus1 : Subsystem
  tag scope: iga_pu_dba_fb_mbafe=global, igb_pu_dbb_fb_mbafe=global, igc_pu_dbc_fb_mbafe=global, isa_pu_dba_fb_mbafe=global, isb_pu_dbb_fb_mbafe=global, isc_pu_dbc_fb_mbafe=global, uga_pu_dba_fb_mbafe=global, ugb_pu_dbb_fb_mbafe=global, ugc_pu_dbc_fb_mbafe=global
  wires:
  [isb_pu_dbb] -> isb_fieldbus/1(is)
  isa_fieldbus/1(is_fb) -> [isa_pu_dba_fb_mbafe]
  [isa_pu_dba] -> isa_fieldbus/1(is)
  isb_fieldbus/1(is_fb) -> [isb_pu_dbb_fb_mbafe]
  [ugb_pu_dbb] -> ugb_fieldbus/1(ug)
  [uga_pu_dba] -> uga_fieldbus/1(ug)
  ugb_fieldbus/1(ug_fb) -> [ugb_pu_dbb_fb_mbafe]
  uga_fieldbus/1(ug_fb) -> [uga_pu_dba_fb_mbafe]
  ugb_fieldbus1/1(ug_fb) -> [ugc_pu_dbc_fb_mbafe]
  [ugc_pu_dbc] -> ugb_fieldbus1/1(ug)
  isc_fieldbus/1(is_fb) -> [isc_pu_dbc_fb_mbafe]
  [isc_pu_dbc] -> isc_fieldbus/1(is)
  [igc_pu_dbc] -> igc_fieldbus/1(is)
  igc_fieldbus/1(is_fb) -> [igc_pu_dbc_fb_mbafe]
  igb_fieldbus/1(is_fb) -> [igb_pu_dbb_fb_mbafe]
  [iga_pu_dba] -> iga_fieldbus/1(is)
  iga_fieldbus/1(is_fb) -> [iga_pu_dba_fb_mbafe]
  [igb_pu_dbb] -> igb_fieldbus/1(is)

== system afe_rst_inv_psm_distributed_control_two_delays/mainboard_afe/voltage_sequence_avg ==
  v_grid_pos_xi : Inport
  v_grid_pos_eta : Inport  Port=2
  v_grid_neg_xi : Inport  Port=3
  v_grid_neg_eta : Inport  Port=4
  Moving Average Filter1 : Subsystem
  Moving Average Filter2 : Subsystem
  Moving Average Filter3 : Subsystem
  Moving Average Filter4 : Subsystem
  v_grid_pos_xi_avg : Outport
  v_grid_pos_eta_avg : Outport  Port=2
  v_grid_neg_xi_avg : Outport  Port=3
  v_grid_neg_eta_avg : Outport  Port=4
  wires:
  [omega_grid_pll] -> Moving Average Filter1/2(In3), Moving Average Filter2/2(In3), Moving Average Filter4/2(In3), Moving Average Filter3/2(In3)
  Moving Average Filter1/1(xi) -> v_grid_pos_xi_avg/1
  v_grid_pos_xi/1 -> Moving Average Filter1/1(In2)
  v_grid_pos_eta/1 -> Moving Average Filter2/1(In2)
  Moving Average Filter2/1(xi) -> v_grid_pos_eta_avg/1
  Moving Average Filter3/1(xi) -> v_grid_neg_xi_avg/1
  v_grid_neg_xi/1 -> Moving Average Filter3/1(In2)
  v_grid_neg_eta/1 -> Moving Average Filter4/1(In2)
  Moving Average Filter4/1(xi) -> v_grid_neg_eta_avg/1

== system afe_rst_inv_psm_distributed_control_two_delays/mainboard_inverter/double_integrator_observer ==
  theta : Inport
  Gain : Gain  Gain=kw
  Gain1 : Gain  Gain=kg
  Gain4 : Gain  Gain=omega_bez
  Gain5 : Gain  Gain=ts_inv
  Gain6 : Gain  Gain=1/omega_bez
  Sum : Sum  Inputs=-+|
  Sum1 : Sum  Inputs=|++
  Sum2 : Sum  Inputs=|++
  Sum8 : Sum  Inputs=++|
  Unit Delay1 : UnitDelay  SampleTime=ts_inv
  Unit Delay2 : UnitDelay  SampleTime=ts_inv
  bounder1 : MATLAB Function  TreatAsAtomicUnit=on  SystemSampleTime=ts_inv
  bounder2 : MATLAB Function  TreatAsAtomicUnit=on  SystemSampleTime=ts_inv
  omega_pu_hat : Outport  VectorParamsAs1DForOutWhenUnconnected=off
  theta_hat : Outport  Port=2  VectorParamsAs1DForOutWhenUnconnected=off
  wires:
  theta/1 -> Sum/2  "theta"
  Sum8/1 -> bounder2/1(u)
  Sum1/1 -> Unit Delay2/1
  Unit Delay2/1 -> omega_pu_hat/1, Sum1/2, Gain5/1
  Sum2/1 -> Sum8/2
  bounder2/1(y) -> Unit Delay1/1
  bounder1/1(y) -> Gain/1, Gain1/1
  Gain5/1 -> Gain4/1
  Sum/1 -> bounder1/1(u)
  Unit Delay1/1 -> Sum2/2, theta_hat/1, Sum/1  "theta_hat"
  Gain/1 -> Gain6/1
  Gain6/1 -> Sum1/1
  Gain4/1 -> Sum8/1
  Gain1/1 -> Sum2/1

== system afe_rst_inv_psm_distributed_control_two_delays/pmsm/synchronous_motor ==
  Bus Selector : BusSelector  OutputSignals=psi_r_alpha (Vs)
  Bus Selector1 : BusSelector  OutputSignals=psi_r_alpha (Vs)
  Bus Selector10 : BusSelector  OutputSignals=uq (V)
  Bus Selector11 : BusSelector  OutputSignals=ud (V)
  Bus Selector12 : BusSelector  OutputSignals=iq (A)
  Bus Selector13 : BusSelector  OutputSignals=id (A)
  Bus Selector2 : BusSelector  OutputSignals=iu (A)
  Bus Selector3 : BusSelector  OutputSignals=iv (A)
  Bus Selector4 : BusSelector  OutputSignals=iw (A)
  Bus Selector5 : BusSelector  OutputSignals=omega_elec (rad/s)
  Bus Selector6 : BusSelector  OutputSignals=phase_elec (rad)
  Bus Selector7 : BusSelector  OutputSignals=pwr_in (kW)
  Bus Selector8 : BusSelector  OutputSignals=pwr_out (kW)
  Bus Selector9 : BusSelector  OutputSignals=torque (Nm)
  Open Circuit : fl_lib/Electrical/Electrical Elements/Open Circuit  v_specify=off  v_priority=None  v=0 V  v_nominal_specify=off  v_nominal_value=1  v_nominal_unit=V
  permanent_magnet_synchronous_machine : permanent_magnet_synchronous_machine/permanent_magnet_synchronous_machine  pp=psm.number_poles  psi_m=psm.psi_m  Lmu=psm.Lmu  La=psm.La_m  Lb=psm.Lb_m  Rs=psm.Rs_m  Jm=psm.Jm_m  b_linear=psm.load_friction_m  b_quadratic=0  h5_percent=0  h7_percent=0  psi_r_u_init=psm.psi_m  psi_r_v_init=-psm.psi_m/2  psi_r_w_init=-psm.psi_m/2  omega_init=0  phase_init=0
  shaft : PMIOPort  Side=Right
  u : PMIOPort  Port=2  Side=Left
  v : PMIOPort  Port=3  Side=Left
  w : PMIOPort  Port=4  Side=Left
  psi_m : PMIOPort  Port=5  Side=Left
  motor_data : Outport
  tag scope: id_psm=global, iq_psm=global, iu_psm=global, iv_psm=global, iw_psm=global, omega_elec_psm=global, psi_r_alpha_psm=global, psi_r_beta_psm=global, pwr_in_psm=global, pwr_out_psm=global, theta_elec_psm=global, torque_load_psm=global, ud_psm=global, uq_psm=global
  wires:
  permanent_magnet_synchronous_machine/1 -> Bus Selector8/1, Bus Selector10/1, Bus Selector11/1, Bus Selector12/1, Bus Selector13/1, Bus Selector9/1, Bus Selector7/1, Bus Selector6/1, Bus Selector5/1, Bus Selector4/1, Bus Selector3/1, Bus Selector2/1, Bus Selector1/1, Bus Selector/1, motor_data/1
  Bus Selector/1 -> [psi_r_alpha_psm]  "<psi_r_alpha (Vs)>"
  Bus Selector1/1 -> [psi_r_beta_psm]  "<psi_r_alpha (Vs)>"
  Bus Selector2/1 -> [iu_psm]  "<iu (A)>"
  Bus Selector3/1 -> [iv_psm]  "<iv (A)>"
  Bus Selector4/1 -> [iw_psm]  "<iw (A)>"
  Bus Selector5/1 -> [omega_elec_psm]  "<omega_elec (rad/s)>"
  Bus Selector6/1 -> [theta_elec_psm]  "<phase_elec (rad)>"
  Bus Selector7/1 -> [pwr_in_psm]  "<pwr_in (kW)>"
  Bus Selector8/1 -> [pwr_out_psm]  "<pwr_out (kW)>"
  Bus Selector9/1 -> [torque_load_psm]  "<torque (Nm)>"
  Bus Selector10/1 -> [uq_psm]  "<uq (V)>"
  Bus Selector11/1 -> [ud_psm]  "<ud (V)>"
  Bus Selector12/1 -> [iq_psm]  "<iq (A)>"
  Bus Selector13/1 -> [id_psm]  "<id (A)>"
  connections:
  permanent_magnet_synchronous_machine/RConn1 -- shaft/RConn1
  permanent_magnet_synchronous_machine/LConn1 -- u/RConn1
  permanent_magnet_synchronous_machine/LConn2 -- v/RConn1
  permanent_magnet_synchronous_machine/LConn3 -- w/RConn1
  permanent_magnet_synchronous_machine/LConn4 -- psi_m/RConn1
  permanent_magnet_synchronous_machine/LConn5 -- Open Circuit/LConn1

== system afe_rst_inv_psm_distributed_control_two_delays/AFE-Modular/afe_leg_a/dclink_measure ==
  Controlled Voltage Source : fl_lib/Electrical/Electrical Sources/Controlled Voltage Source
  Current Sensor1 : fl_lib/Electrical/Electrical Sensors/Current Sensor
  Electrical Reference : fl_lib/Electrical/Electrical Elements/Electrical Reference
  Gain : Gain  Gain=107.5e3
  Gain1 : Gain  Gain=1/Vdc_bez
  Quantizer : Quantizer  QuantizationInterval=VoltageQuantization
  Resistor : fl_lib/Electrical/Electrical Elements/Resistor  R=107.5 kOhm  i_specify=off  i_priority=None  i=0 A  i_nominal_specify=off  i_nominal_value=1  i_nominal_unit=A  v_specify=off  v_priority=None  v=0 V  v_nominal_specify=off  v_nominal_value=1  v_nominal_unit=V
  Saturation : Saturate  UpperLimit=inf  LowerLimit=1
  im_udc : nesl_utility/PS-Simulink Converter  PhysicalDomain=network_engine_domain  SubClassName=ps_output  LeftPortType=input  RightPortType=output  PseudoPeriodic=off  Frequencies=[]  VectorFormat=1-D array  Unit=A  AffineConversion=on
  udc_dba : Scope
      settings: SampleTime=tc  ActiveDisplayYMinimum=667.03043  ActiveDisplayYMaximum=1216.53397  DataLoggingVariableName=ScopeData2
  udc_pu_dba : Scope
      settings: SampleTime=tc  ActiveDisplayYMinimum=1.05238  ActiveDisplayYMaximum=1.19379
  udc : PMIOPort  Side=Left
  tag scope: udc_pu_dba=global
  wires:
  Gain/1 -> udc_dba/1, Saturation/1
  Quantizer/1 -> Gain1/1
  Saturation/1 -> Quantizer/1
  im_udc/1 -> Gain/1
  Gain1/1 -> udc_pu_dba/1, [udc_pu_dba]
  connections:
  udc/RConn1 -- Controlled Voltage Source/RConn1
  Current Sensor1/RConn1 -- im_udc/LConn1
  Current Sensor1/RConn2 -- Electrical Reference/LConn1 -- Controlled Voltage Source/RConn2
  Resistor/RConn1 -- Current Sensor1/LConn1
  Controlled Voltage Source/LConn1 -- Resistor/LConn1

== system afe_rst_inv_psm_distributed_control_two_delays/AFE-Modular/afe_leg_a/driver_board_a ==
  Constant : Constant  Value=Vdc_norm_ref
  current_ctrl : Subsystem
  dq_pll : Subsystem
  iga_dba_estimator : Subsystem
  udc_ctrl : Subsystem
  voltage-current-acquisition : Subsystem
  us_alphabeta_ctrl : Outport
  tag scope: ixi_ref_dba=global
  wires:
  current_ctrl/1(us_alphabeta_ctrl) -> us_alphabeta_ctrl/1
  [udc_pu_dba] -> udc_ctrl/1(udc_pu)
  udc_ctrl/1(i_xi_ref) -> [ixi_ref_dba], current_ctrl/1(i_xi_ref)  "i_xi_ref"
  Constant/1 -> udc_ctrl/2(udc_pu_ref)

== system afe_rst_inv_psm_distributed_control_two_delays/AFE-Modular/afe_leg_a/modulator ==
  us_alphabeta_ctrl : Inport
  Bus Selector : BusSelector  OutputSignals=pwm_u_top,pwm_u_bottom
  Constant1 : Constant
  sv_pwm : Subsystem
  tag scope: afe_mu_bottom=global, afe_mu_top=global
  wires:
  Bus Selector/2 -> [afe_mu_bottom]  "<pwm_u_bottom>"
  us_alphabeta_ctrl/1 -> sv_pwm/1(ab)
  Bus Selector/1 -> [afe_mu_top]  "<pwm_u_top>"
  Constant1/1 -> sv_pwm/2(enable)
  sv_pwm/1(firing_gates) -> Bus Selector/1
